simulink model "gpio"  (R2019a)
settings: Solver=VariableStepAuto  StartTime=0.0  StopTime=10.0  RelTol=1e-3
libraries: xbsIndex_r4 x2
settings Model: Creator=qwerty40  LastModifiedBy=jackh
settings DataIOCC: ReturnWorkspaceOutputs=off
settings DebuggingCC: ArithmeticOperatorsInVariantConditions=warning
settings SFSimCC: SimUseLocalCustomCode=off
settings RTWCC: RTWUseLocalCustomCode=off
settings CodeAppCC: StateflowObjectComments=on

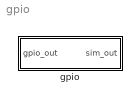
== system gpio ==
  gpio : Subsystem  Tag=xps:gpio  mask(gpio){io_group_params_forwarded=off, io_group=ROACH:led, io_group_real=gpio, io_group_custom=0, io_dir=out, arith_type=Boolean, bitwidth=1, bin_pt=0, bit_index=0, sample_period=1, use_single_ended=off, use_ddr=off, reg_iob=on, reg_clk_phase=0, termination=None, use_iodelay=off}
      mask prompts: io_group_params_forwarded "Have the io_group params been forwarded yet?"; io_group "I/O group"; io_group_real "I/O group"; io_group_custom "Custom I/O group"; io_dir "I/O direction"; arith_type "Data Type"; bitwidth "Data bitwidth"; bin_pt "Data binary point"; bit_index "GPIO bit index"; sample_period "Sample period"; use_single_ended "Use as single-ended"; use_ddr "Use DDR"; reg_iob "Pack register in the pad"; reg_clk_phase "Register clock phase"; termination "Termination method"; use_iodelay "Include IODELAY"
      mask help:
      | GPIO interfaces for CASPER hardware.
      |
      | For usage of LEDs on SKARAB boards, please note that the board will boot into 'BSP mode' by default. To change the control of the Front Panel LEDs to your design, execute the command 'control_front_panel_leds_write()' on your SKARAB CASPERFPGA object via the transport layer.
      |
      | For more information please click help below.
      mask init:
      | gpio_mask;
      mask Help: If you've come here for more help, unfortunately I'm going to direct you to the ska-sa/casperfpga wiki. The documentation at https://github.com/ska-sa/casperfpga/wiki/SKARAB-Front-Panel-LED-Manager outlines the signals that are used to control the SKARAB's Front Panel LEDs by default, and the mechanism by which you can switch control to the DSP Design.
      mask TypeOptions io_group: ROACH:aux0_clk | ROACH:aux1_clk | ROACH:led | ROACH:gpioa | ROACH:gpioa_oe_n | ROACH:gpiob | ROACH:gpiob_oe_n | ROACH:qsh | ROACH:zdok0 | ROACH:zdok1 | ROACH2:aux_clk | ROACH2:led | ROACH2:gpio | ROACH2:qsh | ROACH2:sync_in | ROACH2:sync_out | ROACH2:zdok0 | ROACH2:zdok1 | custom:custom
      mask TypeOptions io_group_real: led | gpio | sync_in | sync_out | zdok0 | zdok1 | aux_clk_diff | custom
      mask Callback io_group_real:
      | if ~isempty(find(strcmp(get_param(gcb, 'io_group_real'), {'zdok0' 'zdok1' 'sync_in' 'sync_out'})))
      |     set_param(gcb, 'MaskEnables', {'off', 'off', 'on','off','on','on','on','on','on','on','on','on','on','on','on','on'});
      | elseif ~isempty(find(strcmp(get_param(gcb, 'io_group_real'), {'custom'})))
      |     set_param(gcb, 'MaskEnables', {'off', 'off', 'on','on','on','on','on','on','on','on','off','on','on','on','on','on'});
      | else
      |     set_param(gcb, 'MaskEnables', {'off', 'off', 'on','off','on','on','on','on','on','on','off','on','on','on','on','on'});
      | end
      mask TypeOptions io_dir: in | out
      mask Callback io_dir:
      | if ~isempty(find(strcmp(get_param(gcb, 'io_group_real'), {'zdok0' 'zdok1' 'sync_in' 'sync_out'})))
      |     set_param(gcb, 'MaskVisibilities', {'off', 'off','on','on','on','on','on','on','on','on','on','on','on','on','on','on'});
      | else
      |     set_param(gcb, 'MaskVisibilities', {'off', 'off','on','on','on','on','on','on','on','on','off','on','on','on','on','on'});
      | end
      mask TypeOptions arith_type: Boolean | Unsigned | Signed  (2's comp)
      mask Callback use_ddr:
      | if strcmp(get_param(gcb,'use_ddr'),'on')
      |     set_param(gcb,'reg_iob','on');
      |     set_param(gcb,'MaskEnables', {'off' 'off' 'on' 'on' 'on' 'on' 'on' 'on' 'on' 'on' 'on' 'on' 'off' 'on' 'on' 'on'});
      | else
      |     set_param(gcb,'MaskEnables', {'off' 'off' 'on' 'on' 'on' 'on' 'on' 'on' 'on' 'on' 'on' 'on' 'on' 'on' 'on' 'on'});
      | end
      mask TypeOptions reg_clk_phase: 0 | 90 | 180 | 270
      mask TypeOptions termination: None | Pullup | Pulldown

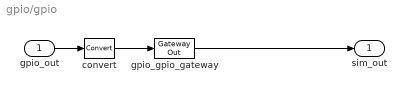
== system gpio/gpio ==
  gpio_out : Inport
  convert : xbsIndex_r4/Convert  gui_display_data_type=Fixed-point  arith_type=Boolean  n_bits=1  bin_pt=0  float_type=Single  exp_bits=8  fraction_bits=24  quantization=Truncate  overflow=Wrap  en=off  latency=1  pipeline=off  dbl_ovrd=off  block_type=convert
  gpio_gpio_gateway : xbsIndex_r4/Gateway Out  inherit_from_input=off  hdl_port=on  rows=1  columns=1  UseAsDAC=off  DACChannel='1'  interface=None  automatic_assignment=on  address_offset=hex2dec('00')  intf_name=''  intf_description=''  timing_constraint=None  locs_specified=off  LOCs={}  io_standard={}  block_type=gatewayout
  sim_out : Outport
  wires:
  gpio_out/1 -> convert/1
  convert/1 -> gpio_gpio_gateway/1
  gpio_gpio_gateway/1 -> sim_out/1
